simulink model "sst_cllc_ttype_inv_discrete"  (R2026b)
settings: Solver=ode23tb  StopTime=simlength  FixedStep=tc  MaxStep=glb_time.tc
values from neighbouring files (symbols this model uses):
  param = sst_cllc_ttype_setup(param)    [init_model.m]
undefined symbols (not defined in the file or in its folder): afe_ctrl, glb_time, grid_emu, hwdata, omega_set, single_phase_inverter_ctrl, sst_num_of_modules
libraries: fl_lib x28, nesl_utility x16, discrete_time_low_pass_filter x4, lithium_ion_battery x2, cllc_dcx x2, dclink_for_three_levels x2, full_bridge_three_level_ttype_ideal_switch_based_model x2, full_bridge_three_level_ttype_mosfet_based_model x2, simulink x2, cstblocks_lti x2, single_phase_three_levels_PWM_modulator x2, dq_vector_pi x2
(part 1 of 3)
settings Model: Creator=LTNBDA  LastModifiedBy=dbagn
settings SolverCC: AutoInsertRateTranBlk=on  SolverResetMethod=Robust  ZeroCrossAlgorithm=Adaptive  ZeroCrossControl=EnableAll
settings DataIOCC: DSMLogging=off  LimitDataPoints=on  MaxDataPoints=1  ReturnWorkspaceOutputs=off  SaveFormat=Array  SaveOutput=off  SaveTime=off  SignalLogging=off  SignalLoggingSaveFormat=ModelDataLogs
settings OptimizationCC: EfficientMapNaN2IntZero=off  LifeSpan=inf  MemsetInitFltsAndDblsToZero=off
settings DebuggingCC: ArithmeticOperatorsInVariantConditions=warning  FcnCallInpInsideContextMsg=warning  MergeDetectMultiDrivingBlocksExec=none  MultiTaskCondExecSysMsg=none  MultiTaskDSMMsg=warning  MultiTaskRateTransMsg=warning  SFNoUnconditionalDefaultTransitionDiag=warning  SFUnexpectedBacktrackingDiag=warning  SaveWithParameterizedLinksMsg=none  SignalResolutionControl=TryResolveAllWithWarning  SolverPrmCheckMsg=warning  StateNameClashWarn=warning
settings HardwareCC: ProdEndianess=Unspecified  ProdEqTarget=off  ProdHWDeviceType=Generic->64-bit Embedded Processor (LP64)  ProdIntDivRoundTo=Undefined  ProdLargestAtomicFloat=None  TargetEndianess=LittleEndian  TargetHWDeviceType=MATLAB Host  TargetIntDivRoundTo=Zero  TargetLongLongMode=on
settings ModelReferenceCC: PropagateSignalLabelsOutOfModel=off
settings SFSimCC: CustomCodeUndefinedFunction=UseInterfaceOnly  SimUseLocalCustomCode=off
settings SFSimCC: SimCustomHeaderCode=|
  | #include "rpi.h"
  | #include "rpi_simulink.h"
  | #include "mavgflt.h"
  | #include "mavgflt_simulink.h"
  | #include "bemf_obsv.h"
  | #include "bemf_obsv_simulink.h"
  | #include "bemf_obsv_load_est.h"
  | #include "bemf_obsv_load_est_simulink.h"
  | #include "dqvector_pi.h"
  | #include "dqvector_pi_simulink.h"
  | #include "sv_pwm_simulink.h"
  | #include "sv_pwm.h"
  | #include "first_harmonic_tracker.h"
  | #include "first_harmonic_tracker_simulink.h"
  | #include "dqpll_thyr.h"
  | #include "dqpll_thyr_simulink.h"
  | #include "dqpll_grid.h"
  | #include "dqpll_grid_simulink.h"
  | #include "sogi_flt.h"
  | #include "sogi_flt_simulink.h"
settings SFSimCC: SimUserIncludeDirs=|
  | include
  | src
settings SFSimCC: SimUserSources=|
  | "mavgflt_simulink.c"
  | "mavgflt.c"
  | "bemf_obsv_simulink.c"
  | "bemf_obsv.c"
  | "bemf_obsv_load_est_simulink.c"
  | "bemf_obsv_load_est.c"
  | "dqvector_pi.c"
  | "dqvector_pi_simulink.c"
  | "sv_pwm_simulink.c"
  | "sv_pwm.c"
  | "first_harmonic_tracker_simulink.c"
  | "first_harmonic_tracker.c"
  | "dqpll_thyr_simulink.c"
  | "dqpll_thyr.c"
  | "dqpll_grid_simulink.c"
  | "dqpll_grid.c"
  | "rpi_simulink.c"
  | "rpi.c"
  | "sogi_flt.c"
  | "sogi_flt_simulink.c"
settings RTWCC: RTWUseLocalCustomCode=off
settings CodeAppCC: StateflowObjectComments=on
settings GRTTargetCC: CombineOutputUpdateFcns=off  GRTInterface=on  TargetLangStandard=C89/C90 (ANSI)
settings ConfigComp: CovExternalEMLEnable=off  CovSaveCumulativeToWorkspaceVar=on  CovSaveSingleToWorkspaceVar=on
settings SimscapeCC: SimscapeNormalizeSystem=off  SimscapeUseEnergyAccounting=off

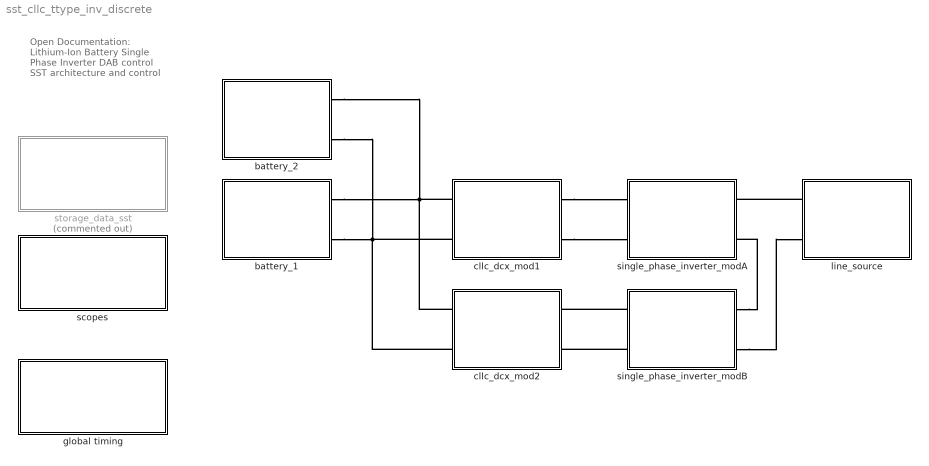
== system sst_cllc_ttype_inv_discrete ==
  note: Open Documentation:
      | Lithium-Ion Battery
      | Single Phase Inverter
      | DAB control
      | SST architecture and control
  battery_1 : Subsystem
  battery_2 : Subsystem
  cllc_dcx_mod1 : Subsystem
  cllc_dcx_mod2 : Subsystem
  global timing : Subsystem
  line_source : Subsystem
  scopes : Subsystem
  single_phase_inverter_modA : Subsystem
  single_phase_inverter_modB : Subsystem
  storage_data_sst : Subsystem  Commented=on
  connections:
  line_source/LConn1 -- single_phase_inverter_modA/RConn1
  battery_1/RConn1 -- cllc_dcx_mod2/LConn1 -- battery_2/RConn1 -- cllc_dcx_mod1/LConn1
  battery_1/RConn2 -- cllc_dcx_mod2/LConn2 -- cllc_dcx_mod1/LConn2 -- battery_2/RConn2
  cllc_dcx_mod1/RConn1 -- single_phase_inverter_modA/LConn1
  cllc_dcx_mod1/RConn2 -- single_phase_inverter_modA/LConn2
  single_phase_inverter_modB/LConn2 -- cllc_dcx_mod2/RConn2
  single_phase_inverter_modB/LConn1 -- cllc_dcx_mod2/RConn1
  single_phase_inverter_modB/RConn1 -- single_phase_inverter_modA/RConn2
  single_phase_inverter_modB/RConn2 -- line_source/LConn2

== system sst_cllc_ttype_inv_discrete/battery_1 ==
  Electrical Reference : fl_lib/Electrical/Electrical Elements/Electrical Reference
  To Workspace14 : ToWorkspace  VariableName=battery_1_data_sim  SampleTime=glb_time.tc
      settings: MaxDataPoints=glb_time.Nc  Decimation=glb_time.decimation_tc
  lithium ion battery : Scope
      settings: ActiveDisplayYMinimum=-70.568782762617388  ActiveDisplayYMaximum=507.60721164031446  DataLoggingVariableName=ScopeData3
  lithium_ion_battery : lithium_ion_battery/lithium_ion_battery  Q=lithium_ion_battery_1.Q  number_of_cells=lithium_ion_battery_1.number_of_cells  E_1=lithium_ion_battery_1.E_1  E0=lithium_ion_battery_1.E0  E1=lithium_ion_battery_1.E1  E2=lithium_ion_battery_1.E2  E3=lithium_ion_battery_1.E3  Elog=lithium_ion_battery_1.Elog  R0=lithium_ion_battery_1.R0  R1=lithium_ion_battery_1.R1  C1=lithium_ion_battery_1.C1  M=lithium_ion_battery_1.M  alpha=lithium_ion_battery_1.alpha  soc_init=lithium_ion_battery_1.soc_init  ts_battery=glb_time.ts_dab  q1Kalman=lithium_ion_battery_1.q1Kalman  q2Kalman=lithium_ion_battery_1.q2Kalman  q3Kalman=lithium_ion_battery_1.q3Kalman  rKalman=lithium_ion_battery_1.rKalman  tc=glb_time.tc  enable_white_noise_m=0  battery_voltage_init_m=param.battery.nominal_battery_voltage_1
  single_phase_ui_measure : Subsystem
  dc(+) : PMIOPort  Side=Right
  dc(-) : PMIOPort  Port=2  Side=Right
  wires:
  lithium_ion_battery/1 -> To Workspace14/1, lithium ion battery/1
  connections:
  single_phase_ui_measure/LConn2 -- Electrical Reference/LConn1 -- lithium_ion_battery/RConn2
  single_phase_ui_measure/RConn1 -- dc(+)/RConn1
  dc(-)/RConn1 -- single_phase_ui_measure/RConn2
  single_phase_ui_measure/LConn1 -- lithium_ion_battery/RConn1

== system sst_cllc_ttype_inv_discrete/battery_2 ==
  To Workspace1 : ToWorkspace  VariableName=battery_2_data_sim  SampleTime=glb_time.tc
      settings: MaxDataPoints=glb_time.Nc  Decimation=glb_time.decimation_tc
  lithium ion battery 2 : Scope
      settings: ActiveDisplayYMinimum=-158.50679627441389  ActiveDisplayYMaximum=914.2862307286149  DataLoggingVariableName=ScopeData3
  lithium_ion_battery : lithium_ion_battery/lithium_ion_battery  Q=lithium_ion_battery_2.Q  number_of_cells=lithium_ion_battery_2.number_of_cells  E_1=lithium_ion_battery_2.E_1  E0=lithium_ion_battery_2.E0  E1=lithium_ion_battery_2.E1  E2=lithium_ion_battery_2.E2  E3=lithium_ion_battery_2.E3  Elog=lithium_ion_battery_2.Elog  R0=lithium_ion_battery_2.R0  R1=lithium_ion_battery_2.R1  C1=lithium_ion_battery_2.C1  M=lithium_ion_battery_2.M  alpha=lithium_ion_battery_2.alpha  soc_init=lithium_ion_battery_2.soc_init  ts_battery=glb_time.ts_dab  q1Kalman=lithium_ion_battery_2.q1Kalman  q2Kalman=lithium_ion_battery_2.q2Kalman  q3Kalman=lithium_ion_battery_2.q3Kalman  rKalman=lithium_ion_battery_2.rKalman  tc=glb_time.tc  enable_white_noise_m=0  battery_voltage_init_m=param.battery.nominal_battery_voltage_2
  single_phase_ui_measure : Subsystem
  udc+ : PMIOPort  Side=Right
  udc- : PMIOPort  Port=2  Side=Right
  wires:
  lithium_ion_battery/1 -> To Workspace1/1, lithium ion battery 2/1
  connections:
  udc-/RConn1 -- single_phase_ui_measure/RConn2
  lithium_ion_battery/RConn1 -- single_phase_ui_measure/LConn1
  single_phase_ui_measure/RConn1 -- udc+/RConn1
  single_phase_ui_measure/LConn2 -- lithium_ion_battery/RConn2

== system sst_cllc_ttype_inv_discrete/cllc_dcx_mod1 ==
  cllc_dcx_mod1 : cllc_dcx/cllc_dcx_mod1  p=param.cllc.p_mod1
  dc1+ : PMIOPort  Side=Left
  dc1- : PMIOPort  Port=2  Side=Left
  dc2+ : PMIOPort  Port=3  Side=Right
  dc2- : PMIOPort  Port=4  Side=Right
  tag scope: cllc_dcx_ctrl_log_mod1=global, cllc_dcx_m_mod1=global
  wires:
  [time_master] -> cllc_dcx_mod1/1
  cllc_dcx_mod1/1 -> [cllc_dcx_m_mod1]
  cllc_dcx_mod1/2 -> [cllc_dcx_ctrl_log_mod1]
  connections:
  cllc_dcx_mod1/RConn2 -- dc2-/RConn1
  cllc_dcx_mod1/LConn2 -- dc1-/RConn1
  cllc_dcx_mod1/RConn1 -- dc2+/RConn1
  cllc_dcx_mod1/LConn1 -- dc1+/RConn1

== system sst_cllc_ttype_inv_discrete/cllc_dcx_mod2 ==
  cllc_dcx_mod1 : cllc_dcx/cllc_dcx_mod1  p=param.cllc.p_mod2
  dc1+ : PMIOPort  Side=Left
  dc1- : PMIOPort  Port=2  Side=Left
  dc2+ : PMIOPort  Port=3  Side=Right
  dc2- : PMIOPort  Port=4  Side=Right
  tag scope: cllc_dcx_ctrl_log_mod2=global, cllc_dcx_m_mod2=global
  wires:
  cllc_dcx_mod1/2 -> [cllc_dcx_ctrl_log_mod2]
  cllc_dcx_mod1/1 -> [cllc_dcx_m_mod2]
  [time_master] -> cllc_dcx_mod1/1
  connections:
  cllc_dcx_mod1/LConn1 -- dc1+/RConn1
  cllc_dcx_mod1/RConn1 -- dc2+/RConn1
  cllc_dcx_mod1/LConn2 -- dc1-/RConn1
  cllc_dcx_mod1/RConn2 -- dc2-/RConn1

== system sst_cllc_ttype_inv_discrete/global timing ==
  Ground_local_time_corr_afe_modA : Ground
  Ground_local_time_corr_afe_modB : Ground
  Ground_local_time_corr_cllc_modA : Ground
  Ground_local_time_corr_cllc_modB : Ground
  Unit Delay{,1..3} (4 alike) : UnitDelay  SampleTime=glb_time.tc
  time_afe_A : Subsystem  mask{k=1}
      mask prompts: k "Time Gain"
      mask Display:
      | disp('time-gen');
      | port_label('input', 1, 'crt');
      | port_label('output', 1, 'tout');
  time_afe_B : Subsystem  mask{k=1}
      mask prompts: k "Time Gain"
      mask Display:
      | disp('time-gen');
      | port_label('input', 1, 'crt');
      | port_label('output', 1, 'tout');
  time_cllc_A : Subsystem  mask{k=1}
      mask prompts: k "Time Gain"
      mask Display:
      | disp('time-gen');
      | port_label('input', 1, 'crt');
      | port_label('output', 1, 'tout');
  time_cllc_B : Subsystem  mask{k=1}
      mask prompts: k "Time Gain"
      mask Display:
      | disp('time-gen');
      | port_label('input', 1, 'crt');
      | port_label('output', 1, 'tout');
  time_master : Subsystem  mask{k=1}
      mask prompts: k "Time Gain"
      mask Display:
      | disp('time-gen');
      | port_label('output', 1, 'tout');
  tag scope: time_afe_module_A=global, time_afe_module_B=global, time_cllc_module_A=global, time_cllc_module_B=global, time_master=global
  wires:
  time_afe_A/1(Out1) -> [time_afe_module_A]
  time_cllc_A/1(Out1) -> [time_cllc_module_A]
  time_cllc_B/1(Out1) -> [time_cllc_module_B]
  time_afe_B/1(Out1) -> [time_afe_module_B]
  time_master/1(Out1) -> [time_master]
  Unit Delay/1 -> time_afe_A/1(correction_time)
  Unit Delay1/1 -> time_cllc_A/1(correction_time)
  Unit Delay2/1 -> time_afe_B/1(correction_time)
  Unit Delay3/1 -> time_cllc_B/1(correction_time)
  Ground_local_time_corr_cllc_modB/1 -> Unit Delay3/1
  Ground_local_time_corr_cllc_modA/1 -> Unit Delay1/1
  Ground_local_time_corr_afe_modB/1 -> Unit Delay2/1
  Ground_local_time_corr_afe_modA/1 -> Unit Delay/1

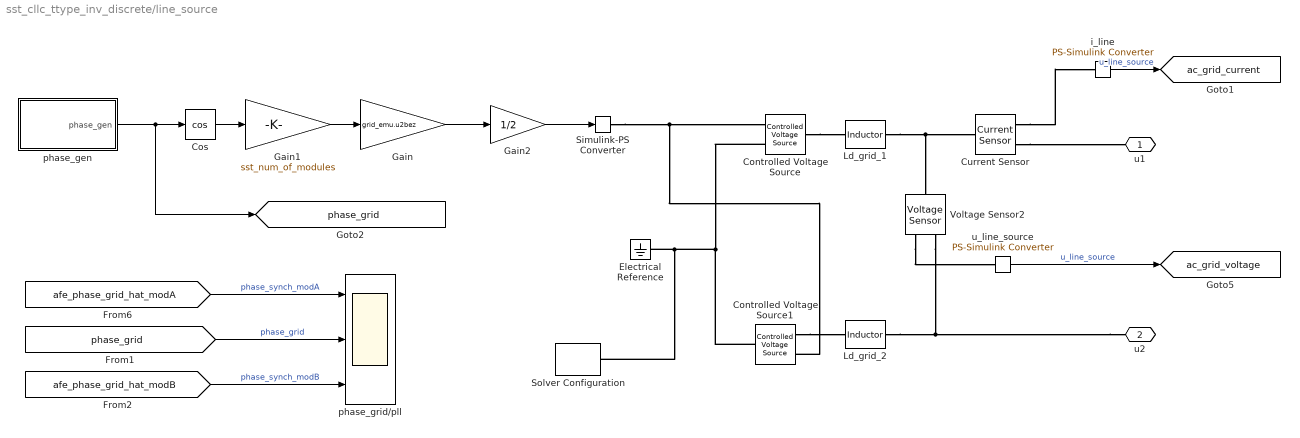
== system sst_cllc_ttype_inv_discrete/line_source ==
  Controlled Voltage Source : fl_lib/Electrical/Electrical Sources/Controlled Voltage Source
  Controlled Voltage Source1 : fl_lib/Electrical/Electrical Sources/Controlled Voltage Source
  Cos : Trigonometry  Operator=cos
  Current Sensor : fl_lib/Electrical/Electrical Sensors/Current Sensor
  Electrical Reference : fl_lib/Electrical/Electrical Elements/Electrical Reference
  Gain : Gain  Gain=grid_emu.u2bez
  Gain1 : Gain  Gain=sst_num_of_modules
  Gain2 : Gain  Gain=1/2
  Ld_grid_1 : fl_lib/Electrical/Electrical Elements/Inductor  l=grid_emu.trafo.Ld2/2 H  r=grid_emu.trafo.Rd2/2 Ohm  g=0 1/Ohm  i_specify=off  i_priority=None  i=0 A  i_nominal_specify=off  i_nominal_value=1  i_nominal_unit=A  v_specify=off  v_priority=None  v=0 V  v_nominal_specify=off  v_nominal_value=1  v_nominal_unit=V  i_L_specify=off  i_L_priority=High  i_L=0 A  i_L_nominal_specify=off  i_L_nominal_value=1  i_L_nominal_unit=A
  Ld_grid_2 : fl_lib/Electrical/Electrical Elements/Inductor  l=grid_emu.trafo.Ld2/2 H  r=grid_emu.trafo.Rd2/2 Ohm  g=0 1/Ohm  i_specify=off  i_priority=None  i=0 A  i_nominal_specify=off  i_nominal_value=1  i_nominal_unit=A  v_specify=off  v_priority=None  v=0 V  v_nominal_specify=off  v_nominal_value=1  v_nominal_unit=V  i_L_specify=off  i_L_priority=High  i_L=0 A  i_L_nominal_specify=off  i_L_nominal_value=1  i_L_nominal_unit=A
  Simulink-PS Converter : nesl_utility/Simulink-PS Converter  PhysicalDomain=network_engine_domain  SubClassName=ps_input  LeftPortType=input  RightPortType=output  PseudoPeriodic=off  Frequencies=[]  NoiseDistribution=none  NoiseParameters=[]  Unit=1  AffineConversion=off  FilteringAndDerivatives=provide  SimscapeFilterOrder=1  InputFilterTimeConstant=0.001  UdotUserProvided=0
  Solver Configuration : nesl_utility/Solver Configuration  PhysicalDomain=network_engine_domain  SubClassName=solver  LeftPortType=input  RightPortType=generic  Tones=[]  Harmonics=[]  SimulateNoise=off  Profile=off  UseLocalSampling=off  EnableSwitchedLinearOptims=on  FrequencyDomain=off  UseCCode=off  RelTol=0.001  AbsTol=0.001  MinStep=1e-09  ToWorkspace=off  RevertToSquareIcSolve=off  NumHomotopyIterations=100  PhasorMode=off  PhasorModeNumHarmonics=1  ConsistencySolver=NEWTON_FTOL  CanonicalOrdering=UNORDERED  OptimizeIntermediates=UNOPTIMIZED  MulticoreSolverChoice=BACKWARD_EULER  IndexReductionMethod=DerivativeReplacement  DoDC=on  ResidualTolerance=1e-3  ConsistencyTolSource=GLOBAL  ConsistencyAbsTol=0.001  ConsistencyRelTol=0.001  ConsistencyTolFactor=0.001  UseLocalSolver=on  LocalSolverChoice=NE_BACKWARD_EULER_ADVANCER  ResolveIndetEquations=on  FunctionEvalNumThread=1  LocalSolverSampleTime=glb_time.tc  DoFixedCost=on  MaxNonlinIter=nonlinear_iterations  MaxModeIter=2  ComputeImpulses=off  ImpulseIterations=2  LinearAlgebra=auto  LinearAlgebraNumThread=0  EquationFormulation=NE_TIME_EF  DelaysMemoryBudget=1024  AutomaticFiltering=on  FilteringTimeConstant=0.001  PartitionStorageMethod=AS_NEEDED  PartitionMemoryBudget=1024  PartitionMethod=BALANCED  MultibodyUseLocalSolver=off  MultibodyLocalSolverChoice=ODE1  MultibodyLocalSolverSampleTime=0.001
  Voltage Sensor2 : fl_lib/Electrical/Electrical Sensors/Voltage Sensor
  i_line : nesl_utility/PS-Simulink Converter  PhysicalDomain=network_engine_domain  SubClassName=ps_output  LeftPortType=input  RightPortType=output  PseudoPeriodic=off  Frequencies=[]  VectorFormat=1-D array  Unit=A  AffineConversion=off
  phase_gen : Subsystem
  phase_grid/pll : Scope  NumInputPorts=3
      settings: ActiveDisplayYMinimum=-3.9269580058491287  ActiveDisplayYMaximum=3.9266955167607471
  u_line_source : nesl_utility/PS-Simulink Converter  PhysicalDomain=network_engine_domain  SubClassName=ps_output  LeftPortType=input  RightPortType=output  PseudoPeriodic=off  Frequencies=[]  VectorFormat=1-D array  Unit=V  AffineConversion=off
  u1 : PMIOPort  Side=Left
  u2 : PMIOPort  Port=2  Side=Left
  tag scope: ac_grid_current=global, ac_grid_voltage=global, phase_grid=global
  wires:
  phase_gen/1(phase_gen) -> Cos/1, [phase_grid]
  Cos/1 -> Gain1/1
  Gain/1 -> Gain2/1
  [afe_phase_grid_hat_modA] -> phase_grid/pll/1  "phase_synch_modA"
  [phase_grid] -> phase_grid/pll/2  "phase_grid"
  u_line_source/1 -> [ac_grid_voltage]  "u_line_source"
  Gain1/1 -> Gain/1
  [afe_phase_grid_hat_modB] -> phase_grid/pll/3  "phase_synch_modB"
  i_line/1 -> [ac_grid_current]  "u_line_source"
  Gain2/1 -> Simulink-PS Converter/1
  connections:
  Simulink-PS Converter/RConn1 -- Controlled Voltage Source1/RConn1 -- Controlled Voltage Source/RConn1
  Voltage Sensor2/RConn1 -- u_line_source/LConn1
  Ld_grid_1/RConn1 -- Current Sensor/LConn1 -- Voltage Sensor2/LConn1
  Solver Configuration/RConn1 -- Electrical Reference/LConn1 -- Controlled Voltage Source/RConn2 -- Controlled Voltage Source1/LConn1
  Controlled Voltage Source/LConn1 -- Ld_grid_1/LConn1
  Current Sensor/RConn2 -- u1/RConn1
  Current Sensor/RConn1 -- i_line/LConn1
  u2/RConn1 -- Ld_grid_2/RConn1 -- Voltage Sensor2/RConn2
  Controlled Voltage Source1/RConn2 -- Ld_grid_2/LConn1

== system sst_cllc_ttype_inv_discrete/scopes ==
  afes current/voltage : Scope  NumInputPorts=4
      settings: ActiveDisplayString=3  ActiveDisplayYMinimum=-169.66254573312608  ActiveDisplayYMaximum=237.83172156728784
  scopes_inv_modA : Subsystem  Commented=on
  scopes_inv_modB : Subsystem  Commented=on
  wires:
  [afe_current_output_modB] -> afes current/voltage/3  "afe_current_output_modB"
  [afe_voltage_output_modB] -> afes current/voltage/4  "afe_voltage_output_modB"
  [afe_voltage_output_modA] -> afes current/voltage/2  "afe_voltage_output_modA"
  [afe_current_output_modA] -> afes current/voltage/1  "afe_current_output_modA"

== system sst_cllc_ttype_inv_discrete/single_phase_inverter_modA ==
  dclink : Subsystem
  output_filter : Subsystem
  single phase afe : Subsystem
      settings: PortSchema="{\"entries\":[{\"content\":{\"sides\":[{\"content\":{\"connectorIds\":[\"LConn1\",\"LConn2\"]},\"type\":\"ConnectorPlacement.EquallySpacedRectSide\",\"uuid\":\"4fcf4fea-d38f-431b-8a91-be3ce9782faf\"},{\"content\":{\"connectorIds\":[\"RConn1\",\"RConn2\",\"RConn3\"],\"side\":\"RIGHT\"},\"type\":\"ConnectorPlacement.EquallySpacedRectSide\",\"uuid\":\"0aa56277-92e9-4e3b-84c7-43398254a4d8\"},{\"content\":{\"connectorIds\":[\"In1\"],\"side\":\"TOP\"},\"type\":\"ConnectorPlacement.EquallySpacedRectSide\",\"uuid\":\"5cd150dc-bcaf-4cd7-b2a8-3db203726730\"}]},\"type\":\"ConnectorPlacement.EquallySpacedConnector\",\"uuid\":\"bf8194c4-c327-4d40-bea4-f1e7617f80b4\"}],\"packageUris\":[\"http://schema.mathworks.com/mf0/Connector/R2020b\"],\"version\":\"1.0\"}"
  single phase inverter control : Subsystem
  uac(+) : PMIOPort  Side=Right
  uac(-) : PMIOPort  Port=2  Side=Right
  udc(+) : PMIOPort  Port=3  Side=Left
  udc(-) : PMIOPort  Port=4  Side=Left
  wires:
  single phase inverter control/1(gate_cmds) -> single phase afe/1(gate_commands)
  connections:
  dclink/RConn1 -- single phase afe/RConn1
  dclink/RConn2 -- single phase afe/RConn2
  dclink/RConn3 -- single phase afe/RConn3
  udc(-)/RConn1 -- dclink/LConn2
  udc(+)/RConn1 -- dclink/LConn1
  single phase afe/LConn1 -- output_filter/LConn1
  uac(+)/RConn1 -- output_filter/RConn1
  single phase afe/LConn2 -- output_filter/LConn2
  output_filter/RConn2 -- uac(-)/RConn1

== system sst_cllc_ttype_inv_discrete/single_phase_inverter_modB ==
  dclink : Subsystem
  output_filter : Subsystem
  single phase afe : Subsystem
      settings: PortSchema="{\"entries\":[{\"content\":{\"sides\":[{\"content\":{\"connectorIds\":[\"LConn1\",\"LConn2\"]},\"type\":\"ConnectorPlacement.EquallySpacedRectSide\",\"uuid\":\"4fcf4fea-d38f-431b-8a91-be3ce9782faf\"},{\"content\":{\"connectorIds\":[\"RConn1\",\"RConn2\",\"RConn3\"],\"side\":\"RIGHT\"},\"type\":\"ConnectorPlacement.EquallySpacedRectSide\",\"uuid\":\"0aa56277-92e9-4e3b-84c7-43398254a4d8\"},{\"content\":{\"connectorIds\":[\"In1\"],\"side\":\"TOP\"},\"type\":\"ConnectorPlacement.EquallySpacedRectSide\",\"uuid\":\"5cd150dc-bcaf-4cd7-b2a8-3db203726730\"}]},\"type\":\"ConnectorPlacement.EquallySpacedConnector\",\"uuid\":\"bf8194c4-c327-4d40-bea4-f1e7617f80b4\"}],\"packageUris\":[\"http://schema.mathworks.com/mf0/Connector/R2020b\"],\"version\":\"1.0\"}"
  single phase inverter control : Subsystem
  uac(+) : PMIOPort  Side=Right
  uac(-) : PMIOPort  Port=2  Side=Right
  udc(+) : PMIOPort  Port=3  Side=Left
  udc(-) : PMIOPort  Port=4  Side=Left
  wires:
  single phase inverter control/1(gate_cmds) -> single phase afe/1(gate_commands)
  connections:
  output_filter/RConn2 -- uac(-)/RConn1
  single phase afe/LConn2 -- output_filter/LConn2
  uac(+)/RConn1 -- output_filter/RConn1
  single phase afe/LConn1 -- output_filter/LConn1
  udc(+)/RConn1 -- dclink/LConn1
  udc(-)/RConn1 -- dclink/LConn2
  dclink/RConn3 -- single phase afe/RConn3
  dclink/RConn2 -- single phase afe/RConn2
  dclink/RConn1 -- single phase afe/RConn1

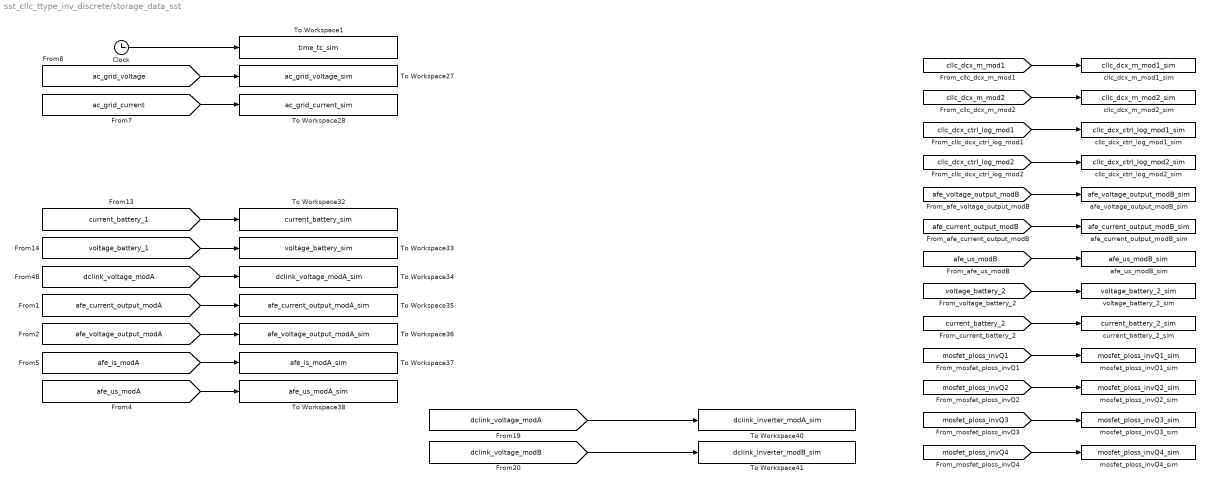
== system sst_cllc_ttype_inv_discrete/storage_data_sst ==
  Clock : Clock
  To Workspace1 : ToWorkspace  VariableName=time_tc_sim  SampleTime=glb_time.tc
      settings: MaxDataPoints=glb_time.Nc  Decimation=glb_time.decimation_tc
  To Workspace27 : ToWorkspace  VariableName=ac_grid_voltage_sim  SampleTime=glb_time.tc
      settings: MaxDataPoints=glb_time.Nc  Decimation=glb_time.decimation_tc
  To Workspace28 : ToWorkspace  VariableName=ac_grid_current_sim  SampleTime=glb_time.tc
      settings: MaxDataPoints=glb_time.Nc  Decimation=glb_time.decimation_tc
  To Workspace32 : ToWorkspace  VariableName=current_battery_sim  SampleTime=glb_time.tc
      settings: MaxDataPoints=glb_time.Nc  Decimation=glb_time.decimation_tc
  To Workspace33 : ToWorkspace  VariableName=voltage_battery_sim  SampleTime=glb_time.tc
      settings: MaxDataPoints=glb_time.Nc  Decimation=glb_time.decimation_tc
  To Workspace34 : ToWorkspace  VariableName=dclink_voltage_modA_sim  SampleTime=glb_time.tc
      settings: MaxDataPoints=glb_time.Nc  Decimation=glb_time.decimation_tc
  To Workspace35 : ToWorkspace  VariableName=afe_current_output_modA_sim  SampleTime=glb_time.tc
      settings: MaxDataPoints=glb_time.Nc  Decimation=glb_time.decimation_tc
  To Workspace36 : ToWorkspace  VariableName=afe_voltage_output_modA_sim  SampleTime=glb_time.tc
      settings: MaxDataPoints=glb_time.Nc  Decimation=glb_time.decimation_tc
  To Workspace37 : ToWorkspace  VariableName=afe_is_modA_sim  SampleTime=glb_time.tc
      settings: MaxDataPoints=glb_time.Nc  Decimation=glb_time.decimation_tc
  To Workspace38 : ToWorkspace  VariableName=afe_us_modA_sim  SampleTime=glb_time.tc
      settings: MaxDataPoints=glb_time.Nc  Decimation=glb_time.decimation_tc
  To Workspace40 : ToWorkspace  VariableName=dclink_inverter_modA_sim  SampleTime=glb_time.tc
      settings: MaxDataPoints=glb_time.Nc  Decimation=glb_time.decimation_tc
  To Workspace41 : ToWorkspace  VariableName=dclink_inverter_modB_sim  SampleTime=glb_time.tc
      settings: MaxDataPoints=glb_time.Nc  Decimation=glb_time.decimation_tc
  afe_current_output_modB_sim : ToWorkspace  VariableName=afe_current_output_modB_sim  SampleTime=glb_time.tc
      settings: MaxDataPoints=glb_time.Nc  Decimation=glb_time.decimation_tc
  afe_us_modB_sim : ToWorkspace  VariableName=afe_us_modB_sim  SampleTime=glb_time.tc
      settings: MaxDataPoints=glb_time.Nc  Decimation=glb_time.decimation_tc
  afe_voltage_output_modB_sim : ToWorkspace  VariableName=afe_voltage_output_modB_sim  SampleTime=glb_time.tc
      settings: MaxDataPoints=glb_time.Nc  Decimation=glb_time.decimation_tc
  cllc_dcx_ctrl_log_mod1_sim : ToWorkspace  VariableName=cllc_dcx_ctrl_log_mod1_sim  SampleTime=glb_time.tc
      settings: MaxDataPoints=glb_time.Nc  Decimation=glb_time.decimation_tc
  cllc_dcx_ctrl_log_mod2_sim : ToWorkspace  VariableName=cllc_dcx_ctrl_log_mod2_sim  SampleTime=glb_time.tc
      settings: MaxDataPoints=glb_time.Nc  Decimation=glb_time.decimation_tc
  cllc_dcx_m_mod1_sim : ToWorkspace  VariableName=cllc_dcx_m_mod1_sim  SampleTime=glb_time.tc
      settings: MaxDataPoints=glb_time.Nc  Decimation=glb_time.decimation_tc
  cllc_dcx_m_mod2_sim : ToWorkspace  VariableName=cllc_dcx_m_mod2_sim  SampleTime=glb_time.tc
      settings: MaxDataPoints=glb_time.Nc  Decimation=glb_time.decimation_tc
  current_battery_2_sim : ToWorkspace  VariableName=current_battery_2_sim  SampleTime=glb_time.tc
      settings: MaxDataPoints=glb_time.Nc  Decimation=glb_time.decimation_tc
  mosfet_ploss_invQ1_sim : ToWorkspace  VariableName=mosfet_ploss_invQ1_sim  SampleTime=glb_time.tc
      settings: MaxDataPoints=glb_time.Nc  Decimation=glb_time.decimation_tc
  mosfet_ploss_invQ2_sim : ToWorkspace  VariableName=mosfet_ploss_invQ2_sim  SampleTime=glb_time.tc
      settings: MaxDataPoints=glb_time.Nc  Decimation=glb_time.decimation_tc
  mosfet_ploss_invQ3_sim : ToWorkspace  VariableName=mosfet_ploss_invQ3_sim  SampleTime=glb_time.tc
      settings: MaxDataPoints=glb_time.Nc  Decimation=glb_time.decimation_tc
  mosfet_ploss_invQ4_sim : ToWorkspace  VariableName=mosfet_ploss_invQ4_sim  SampleTime=glb_time.tc
      settings: MaxDataPoints=glb_time.Nc  Decimation=glb_time.decimation_tc
  voltage_battery_2_sim : ToWorkspace  VariableName=voltage_battery_2_sim  SampleTime=glb_time.tc
      settings: MaxDataPoints=glb_time.Nc  Decimation=glb_time.decimation_tc
  wires:
  Clock/1 -> To Workspace1/1
  [afe_current_output_modA] -> To Workspace35/1
  [afe_voltage_output_modA] -> To Workspace36/1
  [afe_is_modA] -> To Workspace37/1
  [afe_us_modA] -> To Workspace38/1
  [voltage_battery_1] -> To Workspace33/1
  [current_battery_1] -> To Workspace32/1
  [dclink_voltage_modA] -> To Workspace34/1
  [ac_grid_voltage] -> To Workspace27/1
  [ac_grid_current] -> To Workspace28/1
  [dclink_voltage_modA] -> To Workspace40/1
  [dclink_voltage_modB] -> To Workspace41/1
  [cllc_dcx_m_mod1] -> cllc_dcx_m_mod1_sim/1
  [cllc_dcx_m_mod2] -> cllc_dcx_m_mod2_sim/1
  [cllc_dcx_ctrl_log_mod1] -> cllc_dcx_ctrl_log_mod1_sim/1
  [cllc_dcx_ctrl_log_mod2] -> cllc_dcx_ctrl_log_mod2_sim/1
  [afe_voltage_output_modB] -> afe_voltage_output_modB_sim/1
  [afe_current_output_modB] -> afe_current_output_modB_sim/1
  [afe_us_modB] -> afe_us_modB_sim/1
  [voltage_battery_2] -> voltage_battery_2_sim/1
  [current_battery_2] -> current_battery_2_sim/1
  [mosfet_ploss_invQ1] -> mosfet_ploss_invQ1_sim/1
  [mosfet_ploss_invQ2] -> mosfet_ploss_invQ2_sim/1
  [mosfet_ploss_invQ3] -> mosfet_ploss_invQ3_sim/1
  [mosfet_ploss_invQ4] -> mosfet_ploss_invQ4_sim/1

== system sst_cllc_ttype_inv_discrete/battery_1/single_phase_ui_measure ==
  Bus Creator : BusCreator  Inputs=2
  Current Sensor : fl_lib/Electrical/Electrical Sensors/Current Sensor
  Selector : Selector  InputPortWidth=2  IndexOptions=Index vector (dialog)  Indices=2  OutputSizes=1  RuntimeRangeChecks=off
  Selector1 : Selector  InputPortWidth=2  IndexOptions=Index vector (dialog)  Indices=1  OutputSizes=1  RuntimeRangeChecks=off
  Voltage Sensor : fl_lib/Electrical/Electrical Sensors/Voltage Sensor
  battery_1_data : Scope  NumInputPorts=2
      settings: SampleTime=glb_time.tc  ActiveDisplayYMinimum=-325.87342993400324  ActiveDisplayYMaximum=408.02561963983692  DataLoggingVariableName=ScopeData2
  iph : nesl_utility/PS-Simulink Converter  PhysicalDomain=network_engine_domain  SubClassName=ps_output  LeftPortType=input  RightPortType=output  PseudoPeriodic=off  Frequencies=[]  VectorFormat=1-D array  Unit=A  AffineConversion=off
  uph : nesl_utility/PS-Simulink Converter  PhysicalDomain=network_engine_domain  SubClassName=ps_output  LeftPortType=input  RightPortType=output  PseudoPeriodic=off  Frequencies=[]  VectorFormat=1-D array  Unit=V  AffineConversion=off
  Udc(+) : PMIOPort  Side=Left
  udc(+) : PMIOPort  Port=2  Side=Right
  Udc(-) : PMIOPort  Port=3  Side=Left
  udc(-) : PMIOPort  Port=4  Side=Right
  tag scope: current_battery_1=global, voltage_battery_1=global
  wires:
  Bus Creator/1 -> Selector/1, Selector1/1  "ui_data"
  iph/1 -> Bus Creator/1  "iph"
  uph/1 -> Bus Creator/2  "uph"
  Selector1/1 -> [current_battery_1], battery_1_data/1  "current_battery"
  Selector/1 -> battery_1_data/2, [voltage_battery_1]  "voltage_battery"
  connections:
  iph/LConn1 -- Current Sensor/RConn1
  Voltage Sensor/LConn1 -- Current Sensor/LConn1 -- Udc(+)/RConn1
  Current Sensor/RConn2 -- udc(+)/RConn1
  Voltage Sensor/RConn1 -- uph/LConn1
  Voltage Sensor/RConn2 -- Udc(-)/RConn1 -- udc(-)/RConn1

== system sst_cllc_ttype_inv_discrete/battery_2/single_phase_ui_measure ==
  Bus Creator : BusCreator  Inputs=2
  Current Sensor : fl_lib/Electrical/Electrical Sensors/Current Sensor
  Selector : Selector  InputPortWidth=2  IndexOptions=Index vector (dialog)  Indices=2  OutputSizes=1  RuntimeRangeChecks=off
  Selector1 : Selector  InputPortWidth=2  IndexOptions=Index vector (dialog)  Indices=1  OutputSizes=1  RuntimeRangeChecks=off
  Voltage Sensor : fl_lib/Electrical/Electrical Sensors/Voltage Sensor
  dab input modA : Scope  NumInputPorts=2
      settings: SampleTime=glb_time.tc  ActiveDisplayYMinimum=-2492.3665733515445  ActiveDisplayYMaximum=22431.200102395629  DataLoggingVariableName=ScopeData2
  iph : nesl_utility/PS-Simulink Converter  PhysicalDomain=network_engine_domain  SubClassName=ps_output  LeftPortType=input  RightPortType=output  PseudoPeriodic=off  Frequencies=[]  VectorFormat=1-D array  Unit=A  AffineConversion=off
  uph : nesl_utility/PS-Simulink Converter  PhysicalDomain=network_engine_domain  SubClassName=ps_output  LeftPortType=input  RightPortType=output  PseudoPeriodic=off  Frequencies=[]  VectorFormat=1-D array  Unit=V  AffineConversion=off
  Udc(+) : PMIOPort  Side=Left
  udc(+) : PMIOPort  Port=2  Side=Right
  Udc(-) : PMIOPort  Port=3  Side=Left
  udc(-) : PMIOPort  Port=4  Side=Right
  tag scope: current_battery_2=global, voltage_battery_2=global
  wires:
  Selector/1 -> [voltage_battery_2], dab input modA/2  "voltage_battery"
  Selector1/1 -> dab input modA/1, [current_battery_2]  "current_battery"
  uph/1 -> Bus Creator/2  "uph"
  iph/1 -> Bus Creator/1  "iph"
  Bus Creator/1 -> Selector1/1, Selector/1  "ui_data"
  connections:
  udc(-)/RConn1 -- Udc(-)/RConn1 -- Voltage Sensor/RConn2
  Voltage Sensor/RConn1 -- uph/LConn1
  Current Sensor/RConn2 -- udc(+)/RConn1
  Udc(+)/RConn1 -- Current Sensor/LConn1 -- Voltage Sensor/LConn1
  iph/LConn1 -- Current Sensor/RConn1

== system sst_cllc_ttype_inv_discrete/global timing/time_afe_A ==
  correction_time : Inport
  Constant : Constant
  Gain : Gain  Gain=k
  Product : Product
  Sum : Sum  Inputs=|++
  time_1 : Clock
  Out1 : Outport
  wires:
  time_1/1 -> Gain/1
  Gain/1 -> Product/1
  Product/1 -> Out1/1
  correction_time/1 -> Sum/1
  Sum/1 -> Product/2
  Constant/1 -> Sum/2

== system sst_cllc_ttype_inv_discrete/global timing/time_afe_B ==
  correction_time : Inport
  Constant : Constant
  Gain : Gain  Gain=k
  Product : Product
  Sum : Sum  Inputs=|++
  time_1 : Clock
  Out1 : Outport
  wires:
  time_1/1 -> Gain/1
  Gain/1 -> Product/1
  Product/1 -> Out1/1
  correction_time/1 -> Sum/1
  Constant/1 -> Sum/2
  Sum/1 -> Product/2

== system sst_cllc_ttype_inv_discrete/global timing/time_cllc_A ==
  correction_time : Inport
  Constant : Constant
  Gain : Gain  Gain=k
  Product : Product
  Sum : Sum  Inputs=|++
  time_1 : Clock
  Out1 : Outport
  wires:
  time_1/1 -> Gain/1
  Gain/1 -> Product/1
  Product/1 -> Out1/1
  correction_time/1 -> Sum/1
  Constant/1 -> Sum/2
  Sum/1 -> Product/2

== system sst_cllc_ttype_inv_discrete/global timing/time_cllc_B ==
  correction_time : Inport
  Constant : Constant
  Gain : Gain  Gain=k
  Product : Product
  Sum : Sum  Inputs=|++
  time_1 : Clock
  Out1 : Outport
  wires:
  time_1/1 -> Gain/1
  Gain/1 -> Product/1
  Product/1 -> Out1/1
  correction_time/1 -> Sum/1
  Constant/1 -> Sum/2
  Sum/1 -> Product/2

== system sst_cllc_ttype_inv_discrete/global timing/time_master ==
  Gain : Gain  Gain=k
  time_1 : Clock
  Out1 : Outport
  wires:
  Gain/1 -> Out1/1
  time_1/1 -> Gain/1

== system sst_cllc_ttype_inv_discrete/line_source/phase_gen ==
  Constant4 : Constant  Value=grid_emu.omega_grid_nom
  Integrator : Integrator
  bounder1 : MATLAB Function  TreatAsAtomicUnit=on
  phase_gen : Outport  VectorParamsAs1DForOutWhenUnconnected=off
  wires:
  Constant4/1 -> Integrator/1
  Integrator/1 -> bounder1/1(u)
  bounder1/1(y) -> phase_gen/1  "grid_emu_phase"

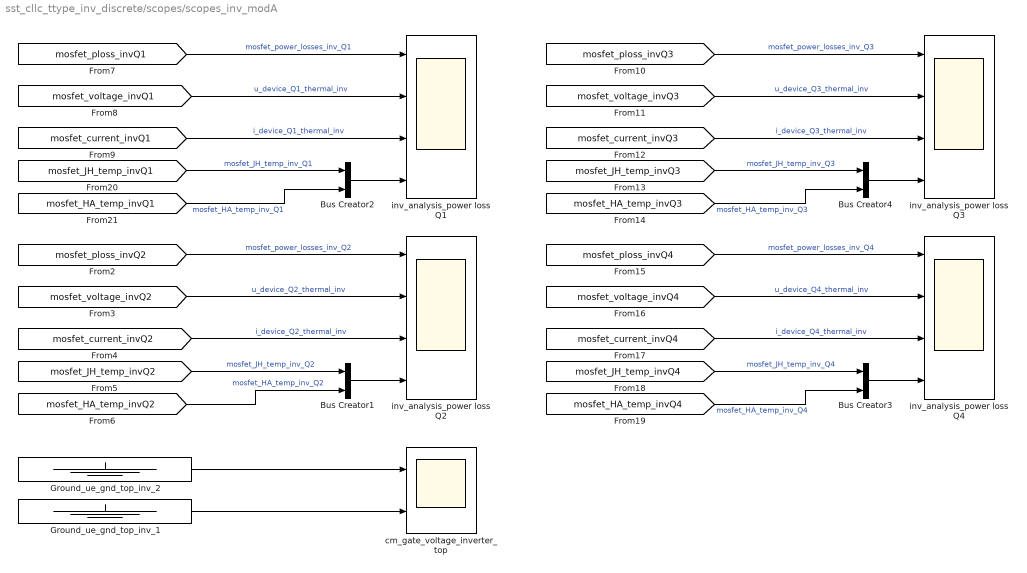
== system sst_cllc_ttype_inv_discrete/scopes/scopes_inv_modA ==
  Bus Creator{1..4} (4 alike) : BusCreator  Inputs=2
  Ground_ue_gnd_top_inv_1 : Ground
  Ground_ue_gnd_top_inv_2 : Ground
  cm_gate_voltage_inverter_top : Scope  NumInputPorts=2
      settings: ActiveDisplayYMinimum=-1089.6954299405313  ActiveDisplayYMaximum=1165.8713445946826  DataLoggingVariableName=ScopeData22
  inv_analysis_power loss Q{1..4} (4 alike) : Scope  NumInputPorts=4
      inv_analysis_power loss Q1 settings: ActiveDisplayYMinimum=252.03887543128099  ActiveDisplayYMaximum=654.5130246681365  DataLoggingVariableName=ScopeData18
      inv_analysis_power loss Q2 settings: ActiveDisplayYMinimum=1215.5585157804567  ActiveDisplayYMaximum=1882.3509853926439  DataLoggingVariableName=ScopeData5
      inv_analysis_power loss Q3 settings: ActiveDisplayYMinimum=1399.7218598743666  ActiveDisplayYMaximum=1614.3940109339064  DataLoggingVariableName=ScopeData16
      inv_analysis_power loss Q4 settings: ActiveDisplayYMinimum=401.80036733196005  ActiveDisplayYMaximum=489.90080295034829  DataLoggingVariableName=ScopeData19
  wires:
  [mosfet_JH_temp_invQ1] -> Bus Creator2/1  "mosfet_JH_temp_inv_Q1"
  [mosfet_voltage_invQ1] -> inv_analysis_power loss Q1/2  "u_device_Q1_thermal_inv"
  [mosfet_current_invQ1] -> inv_analysis_power loss Q1/3  "i_device_Q1_thermal_inv"
  [mosfet_HA_temp_invQ1] -> Bus Creator2/2  "mosfet_HA_temp_inv_Q1"
  Bus Creator2/1 -> inv_analysis_power loss Q1/4
  [mosfet_ploss_invQ1] -> inv_analysis_power loss Q1/1  "mosfet_power_losses_inv_Q1"
  [mosfet_ploss_invQ2] -> inv_analysis_power loss Q2/1  "mosfet_power_losses_inv_Q2"
  Bus Creator1/1 -> inv_analysis_power loss Q2/4
  [mosfet_HA_temp_invQ2] -> Bus Creator1/2  "mosfet_HA_temp_inv_Q2"
  [mosfet_current_invQ2] -> inv_analysis_power loss Q2/3  "i_device_Q2_thermal_inv"
  [mosfet_voltage_invQ2] -> inv_analysis_power loss Q2/2  "u_device_Q2_thermal_inv"
  [mosfet_JH_temp_invQ2] -> Bus Creator1/1  "mosfet_JH_temp_inv_Q2"
  [mosfet_JH_temp_invQ4] -> Bus Creator3/1  "mosfet_JH_temp_inv_Q4"
  [mosfet_voltage_invQ4] -> inv_analysis_power loss Q4/2  "u_device_Q4_thermal_inv"
  [mosfet_current_invQ4] -> inv_analysis_power loss Q4/3  "i_device_Q4_thermal_inv"
  [mosfet_HA_temp_invQ4] -> Bus Creator3/2  "mosfet_HA_temp_inv_Q4"
  Bus Creator3/1 -> inv_analysis_power loss Q4/4
  [mosfet_ploss_invQ4] -> inv_analysis_power loss Q4/1  "mosfet_power_losses_inv_Q4"
  [mosfet_ploss_invQ3] -> inv_analysis_power loss Q3/1  "mosfet_power_losses_inv_Q3"
  Bus Creator4/1 -> inv_analysis_power loss Q3/4
  [mosfet_HA_temp_invQ3] -> Bus Creator4/2  "mosfet_HA_temp_inv_Q3"
  [mosfet_current_invQ3] -> inv_analysis_power loss Q3/3  "i_device_Q3_thermal_inv"
  [mosfet_voltage_invQ3] -> inv_analysis_power loss Q3/2  "u_device_Q3_thermal_inv"
  [mosfet_JH_temp_invQ3] -> Bus Creator4/1  "mosfet_JH_temp_inv_Q3"
  Ground_ue_gnd_top_inv_2/1 -> cm_gate_voltage_inverter_top/1
  Ground_ue_gnd_top_inv_1/1 -> cm_gate_voltage_inverter_top/2

== system sst_cllc_ttype_inv_discrete/scopes/scopes_inv_modB ==
  Ground_i_device_Q1_ideal_inv_modB : Ground
  Ground_u_device_Q1_ideal_inv_modB : Ground
  Ground_udc12_inverter_modB : Ground
  Ground_ue_gnd_bottom_inv_1 : Ground
  Ground_ue_gnd_bottom_inv_2 : Ground
  cm_gate_voltage_inverter_bottom : Scope  NumInputPorts=2
      settings: ActiveDisplayYMinimum=-1241.6958905586757  ActiveDisplayYMaximum=1224.9152234663466  DataLoggingVariableName=ScopeData22
  device_voltage_current_inv Q1 modB : Scope  NumInputPorts=3
      settings: ActiveDisplayYMinimum=-119.06518095025848  ActiveDisplayYMaximum=1054.0032225267662  DataLoggingVariableName=ScopeData20
  wires:
  Ground_ue_gnd_bottom_inv_2/1 -> cm_gate_voltage_inverter_bottom/1
  Ground_ue_gnd_bottom_inv_1/1 -> cm_gate_voltage_inverter_bottom/2
  Ground_u_device_Q1_ideal_inv_modB/1 -> device_voltage_current_inv Q1 modB/1
  Ground_i_device_Q1_ideal_inv_modB/1 -> device_voltage_current_inv Q1 modB/2
  Ground_udc12_inverter_modB/1 -> device_voltage_current_inv Q1 modB/3

== system sst_cllc_ttype_inv_discrete/single_phase_inverter_modA/dclink ==
  Open Circuit : fl_lib/Electrical/Electrical Elements/Open Circuit  v_specify=off  v_priority=None  v=0 V  v_nominal_specify=off  v_nominal_value=1  v_nominal_unit=V
  dclink : dclink_for_three_levels/dclink  Cdc1_m=hwdata.single_phase_inverter.CFi1  Cdc2_m=hwdata.single_phase_inverter.CFi2  Rudc_measure=107e3  Vdc_scale=hwdata.cllc.udc2_bez  Vdc1_m_init=hwdata.cllc.udc2_bez/2  Vdc2_m_init=hwdata.cllc.udc2_bez/2
  references : Subsystem
  Udc(+) : PMIOPort  Side=Right
  np : PMIOPort  Port=2  Side=Right
  Udc(-) : PMIOPort  Port=3  Side=Right
  udc(+) : PMIOPort  Port=4  Side=Left
  udc(-) : PMIOPort  Port=5  Side=Left
  wires:
  dclink/1 -> references/1(m)
  connections:
  Open Circuit/LConn1 -- dclink/RConn2
  udc(+)/RConn1 -- dclink/RConn1
  udc(-)/RConn1 -- dclink/RConn3
  Udc(+)/RConn1 -- dclink/LConn1
  Udc(-)/RConn1 -- dclink/LConn3
  dclink/LConn2 -- np/RConn1

== system sst_cllc_ttype_inv_discrete/single_phase_inverter_modA/output_filter ==
  Capacitor : fl_lib/Electrical/Electrical Elements/Capacitor  c=hwdata.single_phase_inverter.CFu F  r=hwdata.single_phase_inverter.RCFu Ohm  g=0 1/Ohm  i_specify=off  i_priority=None  i=0 A  i_nominal_specify=off  i_nominal_value=1  i_nominal_unit=A  v_specify=off  v_priority=None  v=0 V  v_nominal_specify=off  v_nominal_value=1  v_nominal_unit=V  vc_specify=off  vc_priority=High  vc=0 V  vc_nominal_specify=off  vc_nominal_value=1  vc_nominal_unit=V
  Current Sensor : fl_lib/Electrical/Electrical Sensors/Current Sensor
  Current Sensor1 : fl_lib/Electrical/Electrical Sensors/Current Sensor
  LFu1 : fl_lib/Electrical/Electrical Elements/Inductor  l=hwdata.single_phase_inverter.LFu1 H  r=hwdata.single_phase_inverter.RLFu1 Ohm  g=1e-9 1/Ohm  i_specify=off  i_priority=None  i=0 A  i_nominal_specify=off  i_nominal_value=1  i_nominal_unit=A  v_specify=off  v_priority=None  v=0 V  v_nominal_specify=off  v_nominal_value=1  v_nominal_unit=V  i_L_specify=off  i_L_priority=High  i_L=0 A  i_L_nominal_specify=off  i_L_nominal_value=1  i_L_nominal_unit=A
  LFu2 : fl_lib/Electrical/Electrical Elements/Inductor  l=hwdata.single_phase_inverter.LFu2 H  r=hwdata.single_phase_inverter.RLFu2 Ohm  g=1e-9 1/Ohm  i_specify=off  i_priority=None  i=0 A  i_nominal_specify=off  i_nominal_value=1  i_nominal_unit=A  v_specify=off  v_priority=None  v=0 V  v_nominal_specify=off  v_nominal_value=1  v_nominal_unit=V  i_L_specify=off  i_L_priority=High  i_L=0 A  i_L_nominal_specify=off  i_L_nominal_value=1  i_L_nominal_unit=A
  Voltage Sensor1 : fl_lib/Electrical/Electrical Sensors/Voltage Sensor
  Voltage Sensor2 : fl_lib/Electrical/Electrical Sensors/Voltage Sensor
  iph : nesl_utility/PS-Simulink Converter  PhysicalDomain=network_engine_domain  SubClassName=ps_output  LeftPortType=input  RightPortType=output  PseudoPeriodic=off  Frequencies=[]  VectorFormat=1-D array  Unit=A  AffineConversion=off
  iph1 : nesl_utility/PS-Simulink Converter  PhysicalDomain=network_engine_domain  SubClassName=ps_output  LeftPortType=input  RightPortType=output  PseudoPeriodic=off  Frequencies=[]  VectorFormat=1-D array  Unit=A  AffineConversion=off
  uph1 : nesl_utility/PS-Simulink Converter  PhysicalDomain=network_engine_domain  SubClassName=ps_output  LeftPortType=input  RightPortType=output  PseudoPeriodic=off  Frequencies=[]  VectorFormat=1-D array  Unit=V  AffineConversion=off
  uph2 : nesl_utility/PS-Simulink Converter  PhysicalDomain=network_engine_domain  SubClassName=ps_output  LeftPortType=input  RightPortType=output  PseudoPeriodic=off  Frequencies=[]  VectorFormat=1-D array  Unit=V  AffineConversion=off
  Uac(+) : PMIOPort  Side=Left
  uac(+) : PMIOPort  Port=2  Side=Right
  Uac(-) : PMIOPort  Port=3  Side=Left
  uac(-) : PMIOPort  Port=4  Side=Right
  tag scope: afe_current_output_modA=global, afe_is_modA=global, afe_us_modA=global, afe_voltage_output_modA=global
  wires:
  uph1/1 -> [afe_voltage_output_modA]  "inverter_voltage_output"
  iph/1 -> [afe_current_output_modA]  "inverter_current_output"
  iph1/1 -> [afe_is_modA]  "inverter_is_modA"
  uph2/1 -> [afe_us_modA]  "inverter_us_modA"
  connections:
  Voltage Sensor2/LConn1 -- Current Sensor1/RConn2 -- LFu1/LConn1
  Current Sensor/RConn2 -- uac(+)/RConn1 -- Voltage Sensor1/LConn1
  Voltage Sensor1/RConn2 -- Capacitor/RConn1 -- LFu2/RConn1 -- uac(-)/RConn1
  iph/LConn1 -- Current Sensor/RConn1
  Voltage Sensor1/RConn1 -- uph1/LConn1
  LFu1/RConn1 -- Capacitor/LConn1 -- Current Sensor/LConn1
  Uac(-)/RConn1 -- Voltage Sensor2/RConn2 -- LFu2/LConn1
  iph1/LConn1 -- Current Sensor1/RConn1
  Voltage Sensor2/RConn1 -- uph2/LConn1
  Uac(+)/RConn1 -- Current Sensor1/LConn1

== system sst_cllc_ttype_inv_discrete/single_phase_inverter_modA/single phase afe ==
  gate_commands : Inport
  ideal_switch_based_three_level_inverter_ttype : full_bridge_three_level_ttype_ideal_switch_based_model/ideal_switch_based_three_level_inverter_ttype  Vth=ideal_switch.Vth  Ron=ideal_switch.Rds_on  Vdon_diode=ideal_switch.Vdon_diode  Rdon_diode=ideal_switch.Rdon_diode  Csnubber=ideal_switch.Csnubber  Rsnubber=ideal_switch.Rsnubber
  mosfet_based_three_level_inverter_ttype : full_bridge_three_level_ttype_mosfet_based_model/mosfet_based_three_level_inverter_ttype  Commented=on  Vth_m=mosfet.inv.Vth  Rds_on_m=mosfet.inv.Rds_on  Eon_m=mosfet.inv.Eon  Eoff_m=mosfet.inv.Eoff  Erec_m=mosfet.inv.Err  Ion_sw_loss_m=mosfet.inv.Ion_sw_losses  Voff_sw_loss_m=mosfet.inv.Voff_sw_losses  Vdon_diode_m=mosfet.inv.Vdon_diode  Rdon_diode_m=mosfet.inv.Rdon_diode  rth_mosfet_JH_m=mosfet.inv.Rth_mosfet_JH  rth_mosfet_HA_m=heatsink.Rth_mosfet_HA  Csnubber_m=mosfet.inv.Csnubber  Rsnubber_m=mosfet.inv.Rsnubber  JunctionTermalMass_m=mosfet.inv.JunctionTermalMass  mass_heatsink_m=heatsink.no_weight  specific_heat_m=heatsink.cp  Tambient_m=heatsink.Tambient  DThs_init_m=heatsink.DThs_init  tc_m=glb_time.tc
  references : Subsystem  Commented=on
  uac_out(+) : PMIOPort  Side=Left
  uac_out(-) : PMIOPort  Port=2  Side=Left
  udc(+) : PMIOPort  Port=3  Side=Right
  np : PMIOPort  Port=4  Side=Right
  udc(-) : PMIOPort  Port=5  Side=Right
  wires:
  gate_commands/1 -> mosfet_based_three_level_inverter_ttype/1, ideal_switch_based_three_level_inverter_ttype/1
  mosfet_based_three_level_inverter_ttype/1 -> references/1(m)
  connections:
  ideal_switch_based_three_level_inverter_ttype/LConn2 -- mosfet_based_three_level_inverter_ttype/LConn2 -- uac_out(-)/RConn1
  ideal_switch_based_three_level_inverter_ttype/RConn1 -- mosfet_based_three_level_inverter_ttype/RConn1 -- udc(+)/RConn1
  ideal_switch_based_three_level_inverter_ttype/LConn1 -- mosfet_based_three_level_inverter_ttype/LConn1 -- uac_out(+)/RConn1
  ideal_switch_based_three_level_inverter_ttype/RConn3 -- mosfet_based_three_level_inverter_ttype/RConn3 -- udc(-)/RConn1
  ideal_switch_based_three_level_inverter_ttype/RConn2 -- mosfet_based_three_level_inverter_ttype/RConn2 -- np/RConn1

== system sst_cllc_ttype_inv_discrete/single_phase_inverter_modA/single phase inverter control ==
  acquisition_and_scaling_current : Subsystem  Commented=on
  acquisition_and_scaling_current_with_white_noise : Subsystem
  acquisition_and_scaling_dc_voltage : Subsystem
  acquisition_and_scaling_grid_voltage_ac : Subsystem
  acquisition_and_scaling_voltage : Subsystem
  inverter_current_output_pu_reference : Subsystem
  pwm modulator : Subsystem
  single_phase_inverter_ctrl : Subsystem
  gate_cmds : Outport
  tag scope: afe_phase_grid_hat_modA=global, udq_ctrl_out_modA=global
  wires:
  [afe_is_modA] -> acquisition_and_scaling_current_with_white_noise/1(in)
  pwm modulator/1(gate_cmds) -> gate_cmds/1
  [TRGO_AFE_modA] -> single_phase_inverter_ctrl/Trigger
  [afe_voltage_output_modA] -> acquisition_and_scaling_voltage/1(in)
  single_phase_inverter_ctrl/1(u_ctrl_out) -> pwm modulator/1(vout)
  acquisition_and_scaling_current_with_white_noise/1(out) -> single_phase_inverter_ctrl/2(afe_current_output_pu)  "afe_current_output_pu"
  acquisition_and_scaling_voltage/1(out) -> single_phase_inverter_ctrl/1(afe_voltage_output_pu)  "afe_voltage_output_pu"
  inverter_current_output_pu_reference/1(afe_current_output_pu_reference) -> single_phase_inverter_ctrl/3(afe_current output_pu_reference)  "afe_current_output_pu_reference"
  [dclink_voltage_modA] -> acquisition_and_scaling_dc_voltage/1(in)
  acquisition_and_scaling_dc_voltage/1(out) -> single_phase_inverter_ctrl/4(dclink_voltage_pu)  "dclink_voltage_pu"
  [time_afe_module_A] -> single_phase_inverter_ctrl/5(local_time)
  [ac_grid_voltage] -> acquisition_and_scaling_grid_voltage_ac/1(in)
  acquisition_and_scaling_grid_voltage_ac/1(out) -> single_phase_inverter_ctrl/6(ugrid_pu)  "ug_abc"
  single_phase_inverter_ctrl/2(phase_grid_hat) -> [afe_phase_grid_hat_modA]
  single_phase_inverter_ctrl/3(udq_ctrl_out) -> [udq_ctrl_out_modA]

== system sst_cllc_ttype_inv_discrete/single_phase_inverter_modB/dclink ==
  Open Circuit : fl_lib/Electrical/Electrical Elements/Open Circuit  v_specify=off  v_priority=None  v=0 V  v_nominal_specify=off  v_nominal_value=1  v_nominal_unit=V
  dclink : dclink_for_three_levels/dclink  Cdc1_m=hwdata.single_phase_inverter.CFi1  Cdc2_m=hwdata.single_phase_inverter.CFi2  Rudc_measure=107e3  Vdc_scale=hwdata.cllc.udc2_bez  Vdc1_m_init=hwdata.cllc.udc2_bez/2  Vdc2_m_init=hwdata.cllc.udc2_bez/2
  references : Subsystem
  Udc(+) : PMIOPort  Side=Right
  np : PMIOPort  Port=2  Side=Right
  Udc(-) : PMIOPort  Port=3  Side=Right
  udc(+) : PMIOPort  Port=4  Side=Left
  udc(-) : PMIOPort  Port=5  Side=Left
  wires:
  dclink/1 -> references/1(m)
  connections:
  dclink/LConn2 -- np/RConn1
  Udc(-)/RConn1 -- dclink/LConn3
  Udc(+)/RConn1 -- dclink/LConn1
  udc(-)/RConn1 -- dclink/RConn3
  udc(+)/RConn1 -- dclink/RConn1
  Open Circuit/LConn1 -- dclink/RConn2

== system sst_cllc_ttype_inv_discrete/single_phase_inverter_modB/output_filter ==
  Capacitor : fl_lib/Electrical/Electrical Elements/Capacitor  c=hwdata.single_phase_inverter.CFu F  r=hwdata.single_phase_inverter.RCFu Ohm  g=0 1/Ohm  i_specify=off  i_priority=None  i=0 A  i_nominal_specify=off  i_nominal_value=1  i_nominal_unit=A  v_specify=off  v_priority=None  v=0 V  v_nominal_specify=off  v_nominal_value=1  v_nominal_unit=V  vc_specify=off  vc_priority=High  vc=0 V  vc_nominal_specify=off  vc_nominal_value=1  vc_nominal_unit=V
  Current Sensor : fl_lib/Electrical/Electrical Sensors/Current Sensor
  Current Sensor1 : fl_lib/Electrical/Electrical Sensors/Current Sensor
  LFu1 : fl_lib/Electrical/Electrical Elements/Inductor  l=hwdata.single_phase_inverter.LFu1 H  r=hwdata.single_phase_inverter.RLFu1 Ohm  g=1e-9 1/Ohm  i_specify=off  i_priority=None  i=0 A  i_nominal_specify=off  i_nominal_value=1  i_nominal_unit=A  v_specify=off  v_priority=None  v=0 V  v_nominal_specify=off  v_nominal_value=1  v_nominal_unit=V  i_L_specify=off  i_L_priority=High  i_L=0 A  i_L_nominal_specify=off  i_L_nominal_value=1  i_L_nominal_unit=A
  LFu2 : fl_lib/Electrical/Electrical Elements/Inductor  l=hwdata.single_phase_inverter.LFu2 H  r=hwdata.single_phase_inverter.RLFu2 Ohm  g=1e-9 1/Ohm  i_specify=off  i_priority=None  i=0 A  i_nominal_specify=off  i_nominal_value=1  i_nominal_unit=A  v_specify=off  v_priority=None  v=0 V  v_nominal_specify=off  v_nominal_value=1  v_nominal_unit=V  i_L_specify=off  i_L_priority=High  i_L=0 A  i_L_nominal_specify=off  i_L_nominal_value=1  i_L_nominal_unit=A
  Voltage Sensor1 : fl_lib/Electrical/Electrical Sensors/Voltage Sensor
  Voltage Sensor2 : fl_lib/Electrical/Electrical Sensors/Voltage Sensor
  iph : nesl_utility/PS-Simulink Converter  PhysicalDomain=network_engine_domain  SubClassName=ps_output  LeftPortType=input  RightPortType=output  PseudoPeriodic=off  Frequencies=[]  VectorFormat=1-D array  Unit=A  AffineConversion=off
  iph1 : nesl_utility/PS-Simulink Converter  PhysicalDomain=network_engine_domain  SubClassName=ps_output  LeftPortType=input  RightPortType=output  PseudoPeriodic=off  Frequencies=[]  VectorFormat=1-D array  Unit=A  AffineConversion=off
  uph1 : nesl_utility/PS-Simulink Converter  PhysicalDomain=network_engine_domain  SubClassName=ps_output  LeftPortType=input  RightPortType=output  PseudoPeriodic=off  Frequencies=[]  VectorFormat=1-D array  Unit=V  AffineConversion=off
  uph2 : nesl_utility/PS-Simulink Converter  PhysicalDomain=network_engine_domain  SubClassName=ps_output  LeftPortType=input  RightPortType=output  PseudoPeriodic=off  Frequencies=[]  VectorFormat=1-D array  Unit=V  AffineConversion=off
  Uac(+) : PMIOPort  Side=Left
  uac(+) : PMIOPort  Port=2  Side=Right
  Uac(-) : PMIOPort  Port=3  Side=Left
  uac(-) : PMIOPort  Port=4  Side=Right
  tag scope: afe_current_output_modB=global, afe_is_modB=global, afe_us_modB=global, afe_voltage_output_modB=global
  wires:
  uph2/1 -> [afe_us_modB]  "inverter_us_modA"
  iph1/1 -> [afe_is_modB]  "inverter_is_modA"
  iph/1 -> [afe_current_output_modB]  "inverter_current_output"
  uph1/1 -> [afe_voltage_output_modB]  "inverter_voltage_output"
  connections:
  Uac(+)/RConn1 -- Current Sensor1/LConn1
  Voltage Sensor2/RConn1 -- uph2/LConn1
  iph1/LConn1 -- Current Sensor1/RConn1
  LFu2/LConn1 -- Voltage Sensor2/RConn2 -- Uac(-)/RConn1
  Current Sensor/LConn1 -- Capacitor/LConn1 -- LFu1/RConn1
  Voltage Sensor1/RConn1 -- uph1/LConn1
  iph/LConn1 -- Current Sensor/RConn1
  uac(-)/RConn1 -- LFu2/RConn1 -- Capacitor/RConn1 -- Voltage Sensor1/RConn2
  Voltage Sensor1/LConn1 -- uac(+)/RConn1 -- Current Sensor/RConn2
  LFu1/LConn1 -- Current Sensor1/RConn2 -- Voltage Sensor2/LConn1
